simulink model "semi_steer_kinematic_model"  (R2026a)
settings: Solver=ode4  StopTime=12  FixedStep=0.01
settings Model: Creator=31391  LastModifiedBy=31391

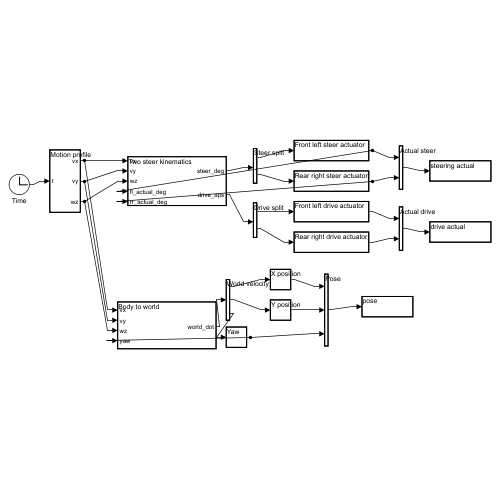
[thumbnail: Simulink's stored preview of the top-level diagram]
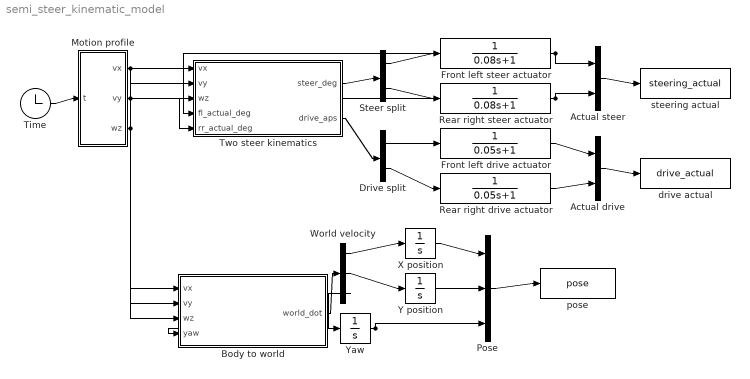
== system semi_steer_kinematic_model ==
  Actual drive : Mux  Inputs=2
  Actual steer : Mux  Inputs=2
  Body to world : MATLAB Function  TreatAsAtomicUnit=on
  Drive split : Demux  Outputs=2
  Front left drive actuator : TransferFcn  Numerator=1  Denominator=[0.05 1]
  Front left steer actuator : TransferFcn  Numerator=1  Denominator=[0.08 1]
  Motion profile : MATLAB Function  TreatAsAtomicUnit=on
  Pose : Mux  Inputs=3
  Rear right drive actuator : TransferFcn  Numerator=1  Denominator=[0.05 1]
  Rear right steer actuator : TransferFcn  Numerator=1  Denominator=[0.08 1]
  Steer split : Demux  Outputs=2
  Time : Clock
  Two steer kinematics : MATLAB Function  TreatAsAtomicUnit=on
  World velocity : Demux  Outputs=3
  X position : Integrator
  Y position : Integrator
  Yaw : Integrator
  drive actual : ToWorkspace  VariableName=drive_actual  SaveFormat=Timeseries  SampleTime=-1
  pose : ToWorkspace  VariableName=pose  SaveFormat=Timeseries  SampleTime=-1
  steering actual : ToWorkspace  VariableName=steering_actual  SaveFormat=Timeseries  SampleTime=-1
  wires:
  Time/1 -> Motion profile/1(t)
  Motion profile/1(vx) -> Two steer kinematics/1(vx), Body to world/1(vx)
  Motion profile/2(vy) -> Two steer kinematics/2(vy), Body to world/2(vy)
  Motion profile/3(wz) -> Two steer kinematics/3(wz), Body to world/3(wz)
  Two steer kinematics/1(steer_deg) -> Steer split/1
  Two steer kinematics/2(drive_aps) -> Drive split/1
  Steer split/1 -> Front left steer actuator/1
  Steer split/2 -> Rear right steer actuator/1
  Front left steer actuator/1 -> Actual steer/1, Two steer kinematics/4(fl_actual_deg)
  Rear right steer actuator/1 -> Actual steer/2, Two steer kinematics/5(rr_actual_deg)
  Actual steer/1 -> steering actual/1
  Drive split/1 -> Front left drive actuator/1
  Drive split/2 -> Rear right drive actuator/1
  Front left drive actuator/1 -> Actual drive/1
  Rear right drive actuator/1 -> Actual drive/2
  Actual drive/1 -> drive actual/1
  Yaw/1 -> Body to world/4(yaw), Pose/3
  Body to world/1(world_dot) -> World velocity/1
  World velocity/1 -> X position/1
  World velocity/2 -> Y position/1
  World velocity/3 -> Yaw/1
  X position/1 -> Pose/1
  Y position/1 -> Pose/2
  Pose/1 -> pose/1

== matlab function semi_steer_kinematic_model/Two steer kinematics ==
  data: vx input; steer_deg output; vy input; wz input; fl_actual_deg input; rr_actual_deg input; drive_aps output
function [steer_deg, drive_aps] = fcn(vx, vy, wz, fl_actual_deg, rr_actual_deg)   
                                                                                 % x points forward, y points left, wz is counterclockwise.                        
                                                                                 wheel_base = 0.344;                                                               
                                                                                 track_width = 0.344;                                                              
                                                                                 wheel_radius = 0.055;                                                             
                                                                                 reduction = 15.76;                                                                
                                                                                 positions = [wheel_base/2, track_width/2; -wheel_base/2, -track_width/2];         
                                                                                 steer_deg = zeros(2,1);                                                           
                                                                                 drive_aps = zeros(2,1);                                                           
                                                                                 actual_deg = [fl_actual_deg; rr_actual_deg];                                      
                                                                                 for i = 1:2                                                                       
                                                                                     vix = vx - wz * positions(i,2);                                               
                                                                                     viy = vy + wz * positions(i,1);                                               
                                                                                     speed = sqrt(vix*vix + viy*viy);                                              
                                                                                     if speed > 0.01                                                               
                                                                                         desired_deg = atan2(viy, vix) * 180 / pi;                                 
                                                                                         error_deg = mod(desired_deg - actual_deg(i) + 180, 360) - 180;            
                                                                                         speed_sign = 1;                                                           
                                                                                         if abs(error_deg) > 90                                                    
                                                                                             error_deg = error_deg - sign(error_deg) * 180;                        
                                                                                             speed_sign = -1;                                                      
                                                                                         end                                                                       
                                                                                         steer_deg(i) = actual_deg(i) + error_deg;                                 
                                                                                         drive_aps(i) = speed_sign * speed * reduction * 360 / (2*pi*wheel_radius);
                                                                                     end                                                                           
                                                                                 end                                                                               
                                                                                 end

== matlab function semi_steer_kinematic_model/Motion profile ==
  data: t input; vx output; vy output; wz output
function [vx, vy, wz] = fcn(t)                        
                                                     % Stop, forward, lateral, rotate, diagonal, then stop.
                                                     vx = 0; vy = 0; wz = 0;                               
                                                     if t >= 2 && t < 4                                    
                                                         vx = 0.60;                                        
                                                     elseif t >= 4 && t < 6                                
                                                         vy = 0.45;                                        
                                                     elseif t >= 6 && t < 8                                
                                                         wz = 0.80;                                        
                                                     elseif t >= 8 && t < 10                               
                                                         vx = 0.50; vy = 0.25; wz = 0.40;                  
                                                     end                                                   
                                                     end

== matlab function semi_steer_kinematic_model/Body to world ==
  data: vx input; world_dot output; vy input; wz input; yaw input
function world_dot = fcn(vx, vy, wz, yaw)                 
                                                         % Ideal body-velocity plant for the first kinematic model.
                                                         c = cos(yaw);                                             
                                                         s = sin(yaw);                                             
                                                         world_dot = [vx*c - vy*s; vx*s + vy*c; wz];               
                                                         end
